simulink model "ProjectRoboticVacuum"  (R2026a)
settings: Solver=VariableStepAuto  StopTime=400  MaxStep=0.01
InitFcn:
  | setupVacuumSim;
StartFcn:
  | learning.simulink.modelCallbacks.startFunction(gcs);
StopFcn:
  | learning.simulink.modelCallbacks.stopFunction(gcs);
model workspace (MAT data in the model file):
  courseObject.course = 'stateflow'
  courseObject.chapter = 7
  courseObject.lesson = 1
  courseObject.section = 2
  courseObject.task = 1
undefined symbols (not defined in the file): axleLength, DiscIntNeverNeededParam, dockX, dockY, initialPos, robotDiam, roomHeight, roomWidth, wheelRadius
libraries: simulink x2, signalChecks x1, SignalEditorBlockLib x1
CloseFcn:
  | learning.simulink.cleanupOnlineTraining;learning.simulink.Application.getInstance().dduxLogMatlabEvent("ModelClosed");
  | if exist('fh','var') && fh.isvalid;close(fh);end;
  | clear('fh','ah','dockHandle','orientationHandle','traceHandle','robotHandle','closefn','existingFigures','figureName','figureTag','lineLength')
  | if exist('fh','var') && fh.isvalid;close(fh);end;
  | clear('fh','ah','dockHandle','orientationHandle','traceHandle','robotHandle','closefn','existingFigures','figureName','figureTag','lineLength')
Description:
  | TrainingCourseModel
settings Model: Creator=PC  LastModifiedBy=PC

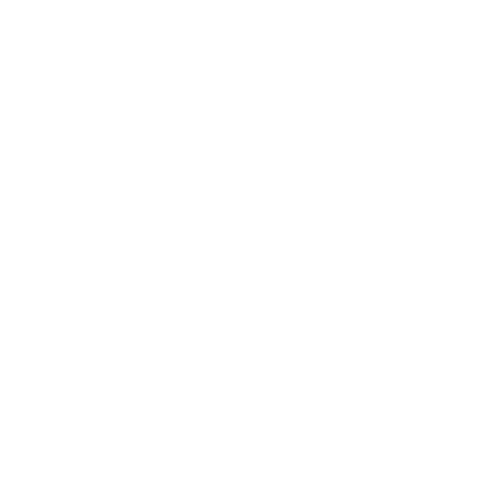
[thumbnail: Simulink's stored preview of the top-level diagram]
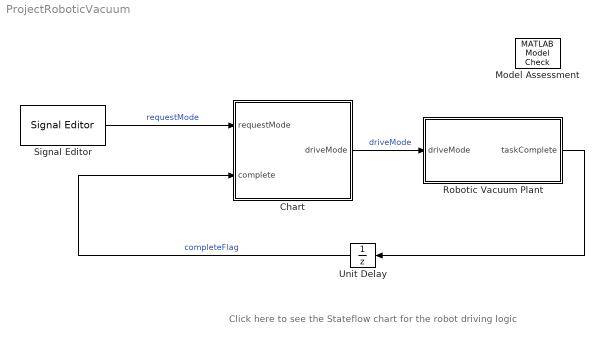
== system ProjectRoboticVacuum ==
  note: Click here to see the Stateflow chart for the robot driving logic
  Chart : Stateflow chart  TreatAsAtomicUnit=on
  Model Assessment : signalChecks/MATLAB Model Check  mlfunc='grader_interaction1_task7'  lesson=0  task=7  pass=1
      settings: AttributesFormatString=|
      | No input required
      | for this task
  Robotic Vacuum Plant : Subsystem
  Signal Editor : SignalEditorBlockLib/Signal Editor  FileName=vacuumScenarios.mat  ActiveScenario=Vacuum  ActiveSignal=Signal  IsBus=off  OutputBusObjectStr=Bus: BusObject  SampleTime=0.1  Interpolate=off  ZeroCross=off  OutputAfterFinalValue=Setting to zero  Unit=inherit  PreserveSignalName=on  ApplySigPropsToAllScenarios=on  ApplySigPropsToAllSignals=off  SignalPropertySource=Dialog parameters
  Unit Delay : UnitDelay  SampleTime=-1
  wires:
  Robotic Vacuum Plant/1(taskComplete) -> Unit Delay/1
  Unit Delay/1 -> Chart/2(complete)  "completeFlag"
  Signal Editor/1 -> Chart/1(requestMode)  "requestMode"
  Chart/1(driveMode) -> Robotic Vacuum Plant/1(driveMode)  "driveMode"

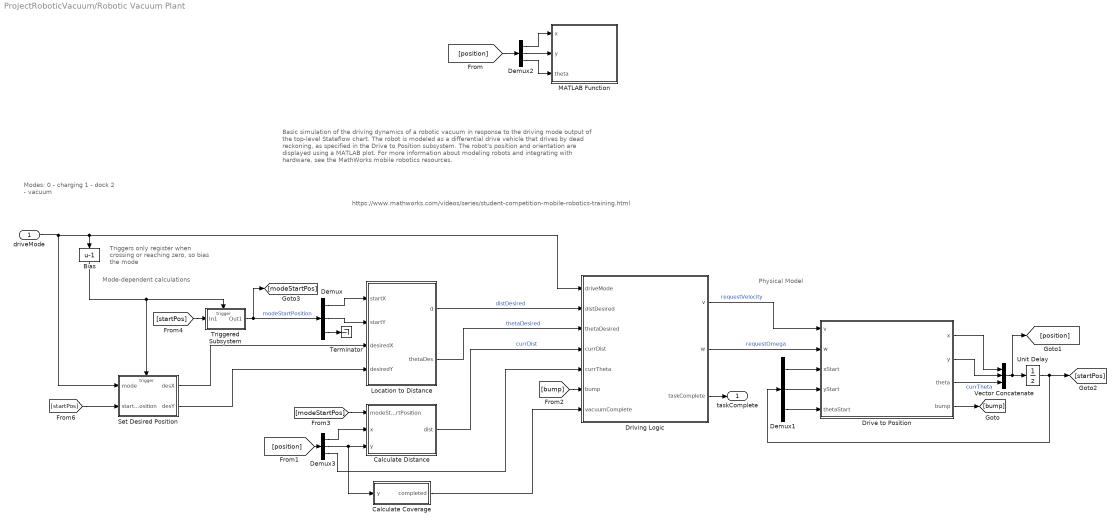
== system ProjectRoboticVacuum/Robotic Vacuum Plant ==
  note: Mode-dependent calculations
  note: Physical Model
  note: https://www.mathworks.com/videos/series/student-competition-mobile-robotics-training.html
  note: Basic simulation of the driving dynamics of a robotic vacuum in response to the driving mode output of the top-level Stateflow chart.
      | The robot is modeled as a differential drive vehicle that drives by dead reckoning, as specified in the Drive to Position subsystem. The robot's position and orientation are displayed using a MATLAB plot.
      |
      | For more information about modeling robots and integrating with hardware, see the MathWorks mobile robotics resources.
  note: Modes:
      | 0 - charging
      | 1 - dock
      | 2 - vacuum
  note: Triggers only register when crossing or reaching zero, so bias the mode
  driveMode : Inport
  Bias : Bias  Bias=-1  SaturateOnIntegerOverflow=off
  Calculate Coverage : Subsystem
  Calculate Distance : Subsystem
  Demux{,1..3} (4 alike) : Demux  Outputs=3
  Drive to Position : Subsystem
  Driving Logic : Stateflow chart  TreatAsAtomicUnit=on
  Location to Distance : Subsystem
  MATLAB Function : MATLAB Function  TreatAsAtomicUnit=on
  Set Desired Position : Subsystem
  Terminator : Terminator
  Triggered Subsystem : Subsystem  TreatAsAtomicUnit=on
  Unit Delay : UnitDelay  InitialCondition=initialPos  SampleTime=-1
  Vector Concatenate : Concatenate  NumInputs=3
  taskComplete : Outport  VectorParamsAs1DForOutWhenUnconnected=off
  wires:
  [modeStartPos] -> Calculate Distance/1(modeStartPosition)
  Demux3/3 -> Driving Logic/5(currTheta)
  Demux3/1 -> Calculate Distance/2(x)
  [position] -> Demux3/1
  Demux3/2 -> Calculate Coverage/1(y), Calculate Distance/3(y)
  Demux2/3 -> MATLAB Function/3(theta)
  Demux2/2 -> MATLAB Function/2(y)
  Demux2/1 -> MATLAB Function/1(x)
  [position] -> Demux2/1
  Calculate Distance/1(dist) -> Driving Logic/4(currDist)  "currDist"
  Demux1/1 -> Drive to Position/3(xStart)
  Demux/2 -> Location to Distance/2(startY)
  [bump] -> Driving Logic/6(bump)
  Driving Logic/3(taskComplete) -> taskComplete/1
  Demux/1 -> Location to Distance/1(startX)
  Drive to Position/4(bump) -> [bump]
  Demux1/3 -> Drive to Position/5(thetaStart)
  Driving Logic/2(w) -> Drive to Position/2(w)  "requestOmega"
  Location to Distance/1(d) -> Driving Logic/2(distDesired)  "distDesired"
  Drive to Position/3(theta) -> Vector Concatenate/3  "currTheta"
  Demux1/2 -> Drive to Position/4(yStart)
  Driving Logic/1(v) -> Drive to Position/1(v)  "requestVelocity"
  Drive to Position/1(x) -> Vector Concatenate/1
  Unit Delay/1 -> [startPos], Demux1/1
  Vector Concatenate/1 -> Unit Delay/1, [position]
  Set Desired Position/1(desX) -> Location to Distance/3(desiredX)
  Set Desired Position/2(desY) -> Location to Distance/4(desiredY)
  driveMode/1 -> Set Desired Position/1(mode), Driving Logic/1(driveMode), Bias/1
  [startPos] -> Set Desired Position/2(startPosition)
  Triggered Subsystem/1(Out1) -> Demux/1, [modeStartPos]  "modeStartPosition"
  Bias/1 -> Triggered Subsystem/Trigger, Set Desired Position/Trigger
  [startPos] -> Triggered Subsystem/1(In1)
  Location to Distance/2(thetaDes) -> Driving Logic/3(thetaDesired)  "thetaDesired"
  Demux/3 -> Terminator/1
  Drive to Position/2(y) -> Vector Concatenate/2
  Calculate Coverage/1(completed) -> Driving Logic/7(vacuumComplete)

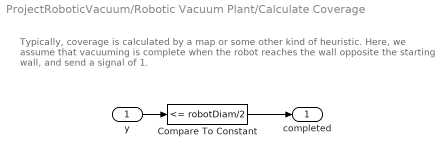
== system ProjectRoboticVacuum/Robotic Vacuum Plant/Calculate Coverage ==
  note: Typically, coverage is calculated by a map or some other kind of heuristic.
      | Here, we assume that vacuuming is complete when the robot reaches the wall opposite the starting wall, and send a signal of 1.
  y : Inport
  Compare To Constant : simulink/Logic and Bit Operations/Compare To Constant  relop=<=  const=robotDiam/2  OutDataTypeStr=boolean
  completed : Outport
  wires:
  y/1 -> Compare To Constant/1
  Compare To Constant/1 -> completed/1

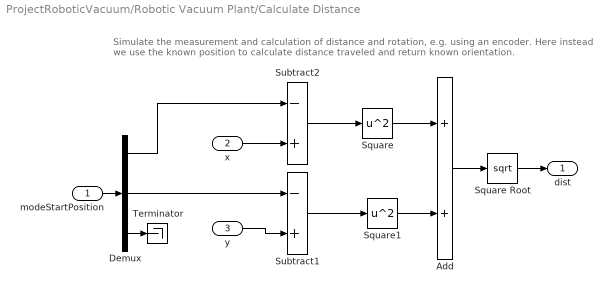
== system ProjectRoboticVacuum/Robotic Vacuum Plant/Calculate Distance ==
  note: Simulate the measurement and calculation of distance and rotation, e.g. using an encoder.
      | Here instead we use the known position to calculate distance traveled and return known orientation.
  modeStartPosition : Inport
  x : Inport  Port=2
  y : Inport  Port=3
  Add : Sum
  Demux : Demux  Outputs=3
  Square : Math  Operator=square  SignedPower=on
  Square Root : Sqrt
  Square1 : Math  Operator=square  SignedPower=on
  Subtract1 : Sum  Inputs=-+
  Subtract2 : Sum  Inputs=-+
  Terminator : Terminator
  dist : Outport  VectorParamsAs1DForOutWhenUnconnected=off
  wires:
  Demux/1 -> Subtract2/1
  x/1 -> Subtract2/2
  Demux/2 -> Subtract1/1
  y/1 -> Subtract1/2
  Subtract2/1 -> Square/1
  Subtract1/1 -> Square1/1
  Square/1 -> Add/1
  Square1/1 -> Add/2
  Add/1 -> Square Root/1
  Square Root/1 -> dist/1
  modeStartPosition/1 -> Demux/1
  Demux/3 -> Terminator/1

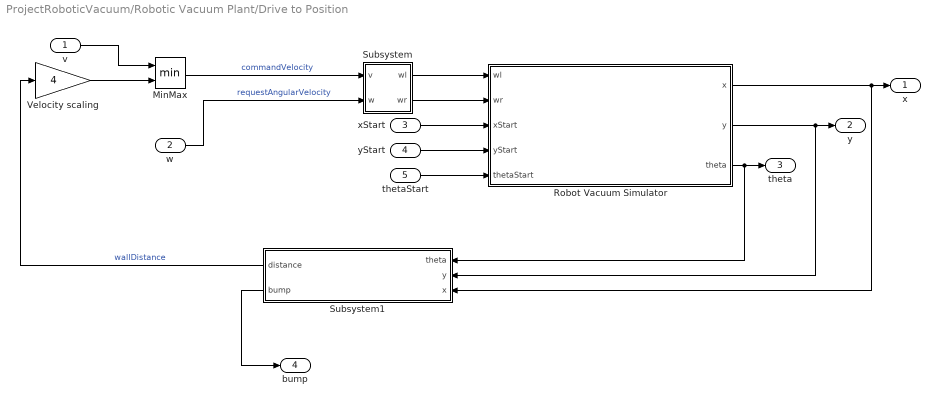
== system ProjectRoboticVacuum/Robotic Vacuum Plant/Drive to Position ==
  v : Inport
  w : Inport  Port=2
  xStart : Inport  Port=3
  yStart : Inport  Port=4
  thetaStart : Inport  Port=5
  MinMax : MinMax  Inputs=2
  Robot Vacuum Simulator : Subsystem  mask(Robot Vacuum Simulator){roomW=roomWidth, roomH=roomHeight, dockX=dockX, dockY=dockY, axleLength=axleLength, wheelR=wheelRadius}
      mask prompts: roomW "Room Width (m)"; roomH "Room Height (m)"; dockX "Dock X (m)"; dockY "Dock Y (m)"; axleLength "Axle Length (m)"; wheelR "Wheel Radius (m)"
      mask help: Model a robot vacuum as a differential drive robot. Simulate its trajectory given prescribed left and right wheel rotation rates (wl, wr) and starting configuration (xStart, yStart, thetaStart).
      mask DialogControl roomProps Prompt: Room Properties
      mask DialogControl robotProps Prompt: Robot Properties
      mask Display: disp('Robot Vacuum Simulator')
  Subsystem : Subsystem  mask(Velocities to wheel angular velocities){axleLength=axleLength, wheelR=wheelRadius}
      mask prompts: axleLength "Axle Length"; wheelR "Wheel Radius"
      mask help: Converts robot linear (v) and angular (w) velocities into left (wl) and right (wr) wheel angular velocities using robot parameters.
  Subsystem1 : Subsystem  mask(Sensor Data Simulator){maxDist=2, minDist=.01}
      mask prompts: maxDist "Maximum sensing distance (m)"; minDist "Minimum sensing distance (m)"
      mask help: Simulate the sensor data from two sensors: an ultrasonic distance sensor measuring distance in meters, and a bump sensor that outputs one when the robot bumps into a wall.
      mask DialogControl Container3 Prompt: Ultrasonic Sensor Properties
      mask Display: disp('Sensor Data Simulator');
  Velocity scaling : Gain  Gain=4
  x : Outport  VectorParamsAs1DForOutWhenUnconnected=off
  y : Outport  Port=2  VectorParamsAs1DForOutWhenUnconnected=off
  theta : Outport  Port=3  VectorParamsAs1DForOutWhenUnconnected=off
  bump : Outport  Port=4  VectorParamsAs1DForOutWhenUnconnected=off
  wires:
  Velocity scaling/1 -> MinMax/2
  w/1 -> Subsystem/2(w)  "requestAngularVelocity"
  Subsystem1/1(distance) -> Velocity scaling/1  "wallDistance"
  Subsystem/1(wl) -> Robot Vacuum Simulator/1(wl)
  Subsystem/2(wr) -> Robot Vacuum Simulator/2(wr)
  xStart/1 -> Robot Vacuum Simulator/3(xStart)
  yStart/1 -> Robot Vacuum Simulator/4(yStart)
  thetaStart/1 -> Robot Vacuum Simulator/5(thetaStart)
  MinMax/1 -> Subsystem/1(v)  "commandVelocity"
  v/1 -> MinMax/1
  Subsystem1/2(bump) -> bump/1
  Robot Vacuum Simulator/3(theta) -> theta/1, Subsystem1/1(theta)
  Robot Vacuum Simulator/2(y) -> y/1, Subsystem1/2(y)
  Robot Vacuum Simulator/1(x) -> x/1, Subsystem1/3(x)

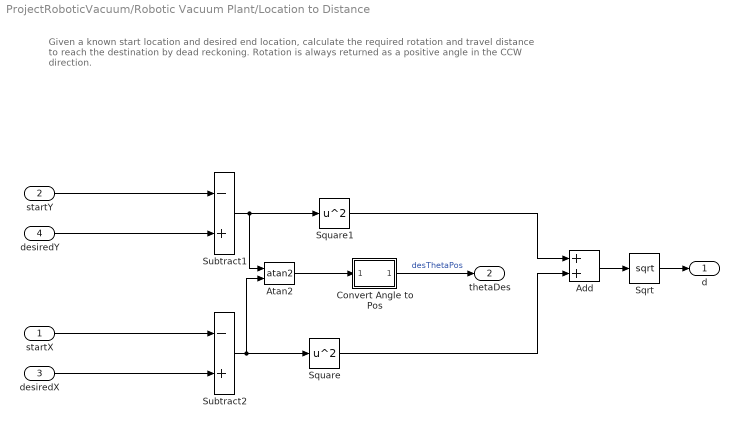
== system ProjectRoboticVacuum/Robotic Vacuum Plant/Location to Distance ==
  note: Given a known start location and desired end location, calculate the required rotation and travel distance to reach the destination by dead reckoning.
      | Rotation is always returned as a positive angle in the CCW direction.
  startX : Inport
  startY : Inport  Port=2
  desiredX : Inport  Port=3
  desiredY : Inport  Port=4
  Add : Sum
  Atan2 : Trigonometry  Operator=atan2
  Convert Angle to Pos : Subsystem
  Sqrt : Sqrt
  Square : Math  Operator=square  SignedPower=on
  Square1 : Math  Operator=square  SignedPower=on
  Subtract1 : Sum  Inputs=-+
  Subtract2 : Sum  Inputs=-+
  d : Outport  VectorParamsAs1DForOutWhenUnconnected=off
  thetaDes : Outport  Port=2  VectorParamsAs1DForOutWhenUnconnected=off
  wires:
  startX/1 -> Subtract2/1
  desiredX/1 -> Subtract2/2
  startY/1 -> Subtract1/1
  desiredY/1 -> Subtract1/2
  Subtract2/1 -> Atan2/2, Square/1
  Square/1 -> Add/2
  Square1/1 -> Add/1
  Add/1 -> Sqrt/1
  Sqrt/1 -> d/1
  Atan2/1 -> Convert Angle to Pos/1(In1)
  Convert Angle to Pos/1(Out1) -> thetaDes/1  "desThetaPos"
  Subtract1/1 -> Square1/1, Atan2/1

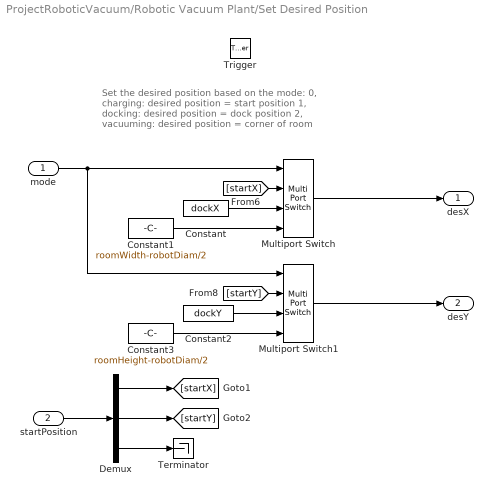
== system ProjectRoboticVacuum/Robotic Vacuum Plant/Set Desired Position ==
  note: Set the desired position based on the mode:
      | 0, charging: desired position = start position
      | 1, docking: desired position = dock position
      | 2, vacuuming: desired position = corner of room
  mode : Inport
  startPosition : Inport  Port=2
  Trigger : TriggerPort  TriggerType=either  VariantControl=Variant  PortDimensions=1
  Constant : Constant  Value=dockX
  Constant1 : Constant  Value=roomWidth-robotDiam/2
  Constant2 : Constant  Value=dockY
  Constant3 : Constant  Value=roomHeight-robotDiam/2
  Demux : Demux  Outputs=3
  Multiport Switch : MultiPortSwitch  DataPortOrder=Zero-based contiguous  zeroidx=on  SaturateOnIntegerOverflow=off  InputSameDT=off
  Multiport Switch1 : MultiPortSwitch  DataPortOrder=Zero-based contiguous  zeroidx=on  SaturateOnIntegerOverflow=off  InputSameDT=off
  Terminator : Terminator
  desX : Outport  VectorParamsAs1DForOutWhenUnconnected=off
  desY : Outport  Port=2  VectorParamsAs1DForOutWhenUnconnected=off
  wires:
  Multiport Switch/1 -> desX/1
  Constant2/1 -> Multiport Switch1/3
  Constant1/1 -> Multiport Switch/4
  [startY] -> Multiport Switch1/2
  Multiport Switch1/1 -> desY/1
  [startX] -> Multiport Switch/2
  mode/1 -> Multiport Switch1/1, Multiport Switch/1
  Constant3/1 -> Multiport Switch1/4
  Constant/1 -> Multiport Switch/3
  startPosition/1 -> Demux/1
  Demux/2 -> [startY]
  Demux/1 -> [startX]
  Demux/3 -> Terminator/1

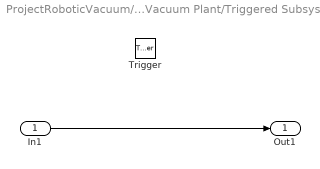
== system ProjectRoboticVacuum/Robotic Vacuum Plant/Triggered Subsystem ==
  In1 : Inport
  Trigger : TriggerPort  TriggerType=either  VariantControl=Variant
  Out1 : Outport  VectorParamsAs1DForOutWhenUnconnected=off
  wires:
  In1/1 -> Out1/1

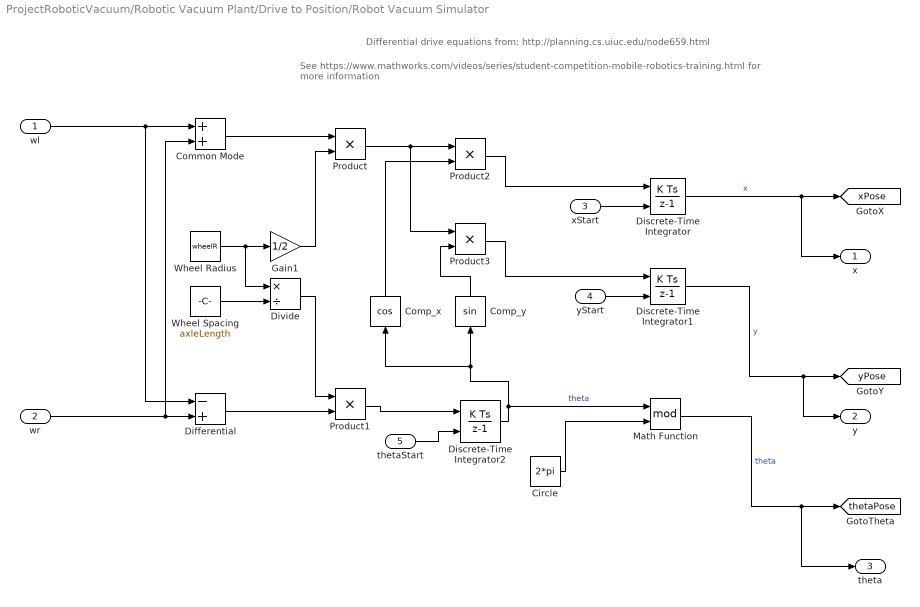
== system ProjectRoboticVacuum/Robotic Vacuum Plant/Drive to Position/Robot Vacuum Simulator ==
  note: Differential drive equations from: http://planning.cs.uiuc.edu/node659.html
  note: See https://www.mathworks.com/videos/series/student-competition-mobile-robotics-training.html for more information
  wl : Inport
  wr : Inport  Port=2
  xStart : Inport  Port=3
  yStart : Inport  Port=4
  thetaStart : Inport  Port=5
  Circle : Constant  Value=2*pi
  Common Mode : Sum
  Comp_x : Trigonometry  Operator=cos
  Comp_y : Trigonometry
  Differential : Sum  Inputs=-+
  Discrete-Time Integrator : DiscreteIntegrator  InitialConditionSource=external  SampleTime=-1  ICPrevOutput=DiscIntNeverNeededParam  ICPrevScaledInput=DiscIntNeverNeededParam
  Discrete-Time Integrator1 : DiscreteIntegrator  InitialConditionSource=external  SampleTime=-1  ICPrevOutput=DiscIntNeverNeededParam  ICPrevScaledInput=DiscIntNeverNeededParam
  Discrete-Time Integrator2 : DiscreteIntegrator  InitialConditionSource=external  SampleTime=-1  ICPrevOutput=DiscIntNeverNeededParam  ICPrevScaledInput=DiscIntNeverNeededParam
  Divide : Product  Inputs=*/
  Gain1 : Gain  Gain=1/2
  Math Function : Math  Operator=mod  SignedPower=on
  Product{,1..3} (4 alike) : Product  RndMeth=Zero
  Wheel Radius : Constant  Value=wheelR
  Wheel Spacing : Constant  Value=axleLength
  x : Outport
  y : Outport  Port=2
  theta : Outport  Port=3
  tag scope: thetaPose=global, xPose=global, yPose=global
  wires:
  Divide/1 -> Product1/1
  Discrete-Time Integrator2/1 -> Math Function/1, Comp_x/1, Comp_y/1  "theta"
  wl/1 -> Common Mode/1, Differential/1
  Product3/1 -> Discrete-Time Integrator1/1
  Comp_x/1 -> Product2/2
  Discrete-Time Integrator/1 -> [xPose], x/1  "x"
  Discrete-Time Integrator1/1 -> [yPose], y/1  "y"
  Wheel Spacing/1 -> Divide/2
  Product1/1 -> Discrete-Time Integrator2/1
  Gain1/1 -> Product/2
  Product/1 -> Product3/1, Product2/1
  Product2/1 -> Discrete-Time Integrator/1
  Comp_y/1 -> Product3/2
  wr/1 -> Common Mode/2, Differential/2
  Wheel Radius/1 -> Divide/1, Gain1/1
  Math Function/1 -> [thetaPose], theta/1  "theta"
  Differential/1 -> Product1/2
  Circle/1 -> Math Function/2
  Common Mode/1 -> Product/1
  thetaStart/1 -> Discrete-Time Integrator2/2
  xStart/1 -> Discrete-Time Integrator/2
  yStart/1 -> Discrete-Time Integrator1/2

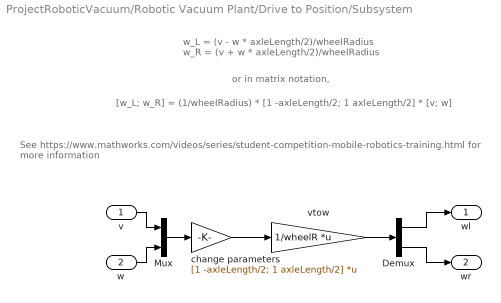
== system ProjectRoboticVacuum/Robotic Vacuum Plant/Drive to Position/Subsystem ==
  note: See https://www.mathworks.com/videos/series/student-competition-mobile-robotics-training.html for more information
  note: [w_L; w_R] = (1/wheelRadius) * [1 -axleLength/2; 1 axleLength/2] * [v; w]
  note: w_L  = (v - w * axleLength/2)/wheelRadius
      | w_R = (v + w * axleLength/2)/wheelRadius
  note: or in matrix notation,
  v : Inport
  w : Inport  Port=2
  Demux : Demux  Outputs=2
  Mux : Mux  Inputs=2
  change parameters : Gain  Gain=[1 -axleLength/2; 1 axleLength/2]  Multiplication=Matrix(K*u)
  vtow : Gain  Gain=1/wheelR  Multiplication=Matrix(K*u)
  wl : Outport  VectorParamsAs1DForOutWhenUnconnected=off
  wr : Outport  Port=2  VectorParamsAs1DForOutWhenUnconnected=off
  wires:
  change parameters/1 -> vtow/1
  w/1 -> Mux/2
  vtow/1 -> Demux/1
  v/1 -> Mux/1
  Demux/1 -> wl/1
  Demux/2 -> wr/1
  Mux/1 -> change parameters/1

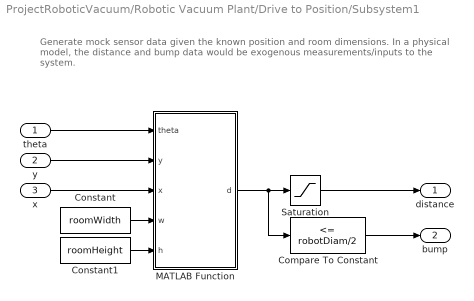
== system ProjectRoboticVacuum/Robotic Vacuum Plant/Drive to Position/Subsystem1 ==
  note: Generate mock sensor data given the known position and room dimensions.
      | In a physical model, the distance and bump data would be exogenous
      | measurements/inputs to the system.
  theta : Inport
  y : Inport  Port=2
  x : Inport  Port=3
  Compare To Constant : simulink/Logic and Bit Operations/Compare To Constant  relop=<=  const=robotDiam/2  OutDataTypeStr=boolean
  Constant : Constant  Value=roomWidth
  Constant1 : Constant  Value=roomHeight
  MATLAB Function : MATLAB Function  TreatAsAtomicUnit=on
  Saturation : Saturate  UpperLimit=maxDist  LowerLimit=minDist
  distance : Outport  VectorParamsAs1DForOutWhenUnconnected=off
  bump : Outport  Port=2  VectorParamsAs1DForOutWhenUnconnected=off
  wires:
  Constant1/1 -> MATLAB Function/5(h)
  Constant/1 -> MATLAB Function/4(w)
  theta/1 -> MATLAB Function/1(theta)
  x/1 -> MATLAB Function/3(x)
  y/1 -> MATLAB Function/2(y)
  Saturation/1 -> distance/1
  MATLAB Function/1(d) -> Compare To Constant/1, Saturation/1
  Compare To Constant/1 -> bump/1

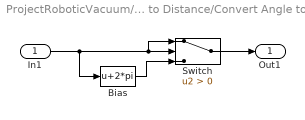
== system ProjectRoboticVacuum/Robotic Vacuum Plant/Location to Distance/Convert Angle to Pos ==
  In1 : Inport
  Bias : Bias  Bias=2*pi  SaturateOnIntegerOverflow=off
  Switch : Switch  Criteria=u2 > Threshold  SaturateOnIntegerOverflow=off  InputSameDT=off
  Out1 : Outport  VectorParamsAs1DForOutWhenUnconnected=off
  wires:
  In1/1 -> Bias/1, Switch/2, Switch/1
  Switch/1 -> Out1/1
  Bias/1 -> Switch/3

== stateflow chart ProjectRoboticVacuum/Chart ==
  settings: updateMethod=DISCRETE  sampleTime=0.1
  state Vacuum
    entry:
    driveMode = 2;
    during:
    SOC = SOC - 1e-5;
  state Off
    entry:
    driveMode = 0;
  state SeekDock
    entry:
    driveMode = 1;
    during:
    SOC = SOC - 1e-5;
  state Charge
    entry:
    driveMode = 0;
    during:
    SOC = SOC + 2e-5;
  (default) -> Off
  Off -> Vacuum [order 1] : [requestMode == 2]
  Vacuum -> SeekDock [order 2] : [requestMode == 1||complete == 1||SOC < 30]
  SeekDock -> Charge [order 2] : [complete == 1]
  Vacuum -> Off [order 1] : [requestMode == -1]
  Off -> SeekDock [order 2] : [requestMode == 1]
  SeekDock -> Off [order 1] : [requestMode == -1]
  Charge -> Off : [SOC >= 97]
  data: requestMode input; driveMode output; complete input; SOC local =100

== matlab function ProjectRoboticVacuum/Robotic Vacuum Plant/MATLAB Function ==
  data: x input; y input; theta input
function plotRobot(x,y,theta)

coder.extrinsic('evalin','plot');



lineLength = .2;

oH = evalin('base','orientationHandle');
rH = evalin('base','robotHandle');

% Find length orientation line
xp = [x x+lineLength*cos(theta)];
yp = [y y+lineLength*sin(theta)];

% Plot robot
set(oH,'xdata',xp,'ydata',yp);
set(rH,'xdata',x,'ydata',y);
drawnow('limitrate')

== matlab function ProjectRoboticVacuum/Robotic Vacuum Plant/Drive to Position/Subsystem1/MATLAB Function ==
  data: theta input; y input; x input; d output; w input; h input
function d = distanceToWall(theta,y,x,w,h)

% Calculate distance to closest wall based on pose

if theta <= pi/2
    dx = w-x;
    dy = h-y;
elseif theta <= pi
    dx = x;
    dy = h-y;
elseif theta <= 3*pi/2
    dx = x;
    dy = y;
else
    dx = w-x;
    dy = y;
end

d = min([dx,dy]);

== stateflow chart ProjectRoboticVacuum/Robotic Vacuum Plant/Driving Logic ==
  settings: updateMethod=DISCRETE  sampleTime=.1
  state Off
  state DriveToPosition
    entry:
    positionReached = 0;
    state PureRotate
      entry:
      v = 0;
      w = 1;
    state PureTranslate
      entry:
      v = 4;
      w = 0;
    state Stop
      entry:
      v = 0;
      w = 0;
      positionReached = 1;
    (default) -> PureRotate
    PureRotate -> PureTranslate : [abs(mod(currTheta,2*pi) - thetaDesired) < 0.05]
    PureTranslate -> Stop : [currDist >= distDesired]
  state TaskComplete
    entry:
    taskComplete = 1;
    exit:
    taskComplete = 0;
  state ZigZag
    % Zig-zag by driving until reaching a wall, then
    % make a U-turn. U-turn direction tracked with
    % local variable, k
    entry:
    k = -1;
    exit:
    v = 0; w = 0;
    state Orient
      entry:
      v = 0;
      w = 0.4;
    state DriveToWall
      entry:
      v = 4;
      w = 0;
    state Uturn
      % Turn 90 degrees, drive forward by dead reckoning, turn 90 degrees
      entry:
      nTurns = 0;
      exit:
      k = k*-1;
      state Rotate
        entry:
        v = 0;
        w = 0.5*k;
        startTheta = currTheta;
        deltaTheta = 0;
        during:
        deltaTheta = abs(currTheta - startTheta);
      state Advance
        entry:
        v = 3;
        w = 0;
      (default) -> Rotate
      Rotate -> Advance : [abs(deltaTheta - (pi/2)) < 0.02]{nTurns = nTurns + 1;}
      Advance -> Rotate : after(100,msec)
    (default) -> Orient
    Orient -> DriveToWall : [abs(currTheta - pi) < 0.02]
    DriveToWall -> Uturn : [bump == 1]
    Uturn -> DriveToWall : [nTurns == 2]
  (default) -> Off
  (junction 64) -> Off
  TaskComplete -> (junction 64) : [after(1,tick)]
  Off -> DriveToPosition : [driveMode ~= 0]
  DriveToPosition -> TaskComplete [order 1] : [driveMode == 0]
  DriveToPosition -> TaskComplete [order 2] : [positionReached == 1 && driveMode == 1]
  ZigZag -> TaskComplete : [vacuumComplete == 1 || driveMode ~= 2]
  DriveToPosition -> ZigZag [order 3] : [positionReached == 1 && driveMode == 2]
  data: driveMode input; distDesired input; thetaDesired input; v output; w output; currDist input; currTheta input; positionReached local; taskComplete output; bump input; k local; nTurns local; vacuumComplete input; deltaTheta local; startTheta local
